simulink model "sm_car"  (R2025a)
settings: Solver=ode23t  StartTime=0.0  StopTime=400  MaxStep=0.4  RelTol=1e-3  AbsTol=1e-3  EnableMultiTasking=on
PreLoadFcn:
  | % Due to usability issue in Repeating Sequence block
  | warning('off','Simulink:Masking:Invalid');
  | 
  | % Eliminate unnecessary warnings in inactive variants
  | % Warnings generated only if you click through inactive variant
  | warning('off','MATLAB:nonExistentField');
  | warning('off','Simulink:Parameters:BlkParamUndefined');
PostLoadFcn:
  | set_param([bdroot '/Vehicle'],'popup_trailer','Off')
  | warning('off','sm:sli:setup:compile:LocalSolverNotSupported')
  | %sm_car_config_maneuver(bdroot,'WOT Braking');
  | sm_car_config_vehicle(bdroot,'false');
  | sm_car_config_logging(bdroot);
InitFcn:
  | sm_car_config_camera;
  | Vehicle = sm_car_vehcfg_checkConfig(Vehicle);
  | sm_car_check_tire_model(bdroot);
StartFcn:
  | tic;
StopFcn:
  | Elapsed_Sim_Time = toc;
  | % disp(['Elapsed Sim Time = ' num2str(Elapsed_Sim_Time)]);
undefined symbols (not defined in the file): Axle1D, AxleIn, Camera, Control, Driver, Free, Init, Maneuver, Pedal, RaceFix, RaceSpin, Scene, ShaftL1, ShaftL2, ShaftR1, ShaftR2, Soft, Stiff, Visual, X, xy_data_car_side, Y, Z
libraries: sm_lib x1546, nesl_utility x528, fl_lib x480, SimscapeFluids_lib x61, sdl_lib x49, simulink x29, ee_lib x7, simulink_extras x6, Linkage_Systems x4, Tire_1x2x x4, AntiRollBar_Systems x2, Linkage_Decoupled x2
(part 6 of 79)

== system sm_car/World/Scene/CRG Hockenheim ==
  Finish Line : Subsystem  mask{post_h=geometry.finish_line.post.height, post_r=geometry.finish_line.post.radius, line_w=geometry.finish_line.post.separation, post_clr=geometry.finish_line.post.clr, post_opc=geometry.finish_line.post.opc, offset_xyz=geometry.finish_line.offset.xyz, offset_yaw=geometry.finish_line.offset.yaw, offset_pitch=geometry.finish_line.offset.pitch, offset_roll=geometry.finish_line.offset.roll}
      mask prompts: post_h "Post Height (m)"; post_r "Post Radius (m)"; line_w "Post Separation (m)"; post_clr "Post Color [R G B] (0-1)"; post_opc "Post Opacity (0-1)"; offset_xyz "Line Offset [x y z] (m)"; offset_yaw "Line Orientation yaw (rad)"; offset_pitch "Line Orientation pitch (rad)"; offset_roll "Line Orientation roll (rad)"
  Ground : Ground
  STL Geometry Centerline : Subsystem  mask{stl_file=geometry.centerline.filename, stl_units=geometry.centerline.fileunits, stl_clr=geometry.centerline.clr, stl_opc=geometry.centerline.opc, stl_x=geometry.centerline.x, stl_y=geometry.centerline.y, stl_z=geometry.centerline.z, stl_yaw=geometry.centerline.yaw, stl_pitch=geometry.centerline.pitch, stl_roll=geometry.centerline.roll}
      mask prompts: stl_file "CAD File"; stl_units "Units"; stl_clr "Color [R G B]"; stl_opc "Opacity (0-1)"; stl_x "Offset x (m)"; stl_y "Offset y (m)"; stl_z "Offset z (m)"; stl_yaw "Offset yaw (rad)"; stl_pitch "Offset pitch (rad)"; stl_roll "Offset roll (rad)"
      mask init:
      | set_param([gcb '/Geometry'],'ExtGeomFileName',stl_file);
      | set_param([gcb '/Geometry'],'ExtGeomFileUnits',stl_units);
  STL Geometry Road : Subsystem  mask{stl_file=geometry.filename, stl_units=geometry.fileunits, stl_clr=geometry.clr, stl_opc=geometry.opc, stl_x=geometry.x, stl_y=geometry.y, stl_z=geometry.z, stl_yaw=geometry.yaw, stl_pitch=geometry.pitch, stl_roll=geometry.roll}
      mask prompts: stl_file "CAD File"; stl_units "Units"; stl_clr "Color [R G B]"; stl_opc "Opacity (0-1)"; stl_x "Offset x (m)"; stl_y "Offset y (m)"; stl_z "Offset z (m)"; stl_yaw "Offset yaw (rad)"; stl_pitch "Offset pitch (rad)"; stl_roll "Offset roll (rad)"
      mask init:
      | set_param([gcb '/Geometry'],'ExtGeomFileName',stl_file);
      | set_param([gcb '/Geometry'],'ExtGeomFileUnits',stl_units);
  W : PMIOPort  Side=Left
  Obs : Outport  VectorParamsAs1DForOutWhenUnconnected=off
  wires:
  Ground/1 -> Obs/1
  connections:
  STL Geometry Centerline/RConn1 -- Finish Line/LConn1 -- W/RConn1 -- STL Geometry Road/RConn1

== system sm_car/World/Scene/CRG Hockenheim F ==
  Finish Line : Subsystem  mask{post_h=geometry.finish_line.post.height, post_r=geometry.finish_line.post.radius, line_w=geometry.finish_line.post.separation, post_clr=geometry.finish_line.post.clr, post_opc=geometry.finish_line.post.opc, offset_xyz=geometry.finish_line.offset.xyz, offset_yaw=geometry.finish_line.offset.yaw, offset_pitch=geometry.finish_line.offset.pitch, offset_roll=geometry.finish_line.offset.roll}
      mask prompts: post_h "Post Height (m)"; post_r "Post Radius (m)"; line_w "Post Separation (m)"; post_clr "Post Color [R G B] (0-1)"; post_opc "Post Opacity (0-1)"; offset_xyz "Line Offset [x y z] (m)"; offset_yaw "Line Orientation yaw (rad)"; offset_pitch "Line Orientation pitch (rad)"; offset_roll "Line Orientation roll (rad)"
  Ground : Ground
  STL Geometry Centerline : Subsystem  mask{stl_file=geometry.centerline.filename, stl_units=geometry.centerline.fileunits, stl_clr=geometry.centerline.clr, stl_opc=geometry.centerline.opc, stl_x=geometry.centerline.x, stl_y=geometry.centerline.y, stl_z=geometry.centerline.z, stl_yaw=geometry.centerline.yaw, stl_pitch=geometry.centerline.pitch, stl_roll=geometry.centerline.roll}
      mask prompts: stl_file "CAD File"; stl_units "Units"; stl_clr "Color [R G B]"; stl_opc "Opacity (0-1)"; stl_x "Offset x (m)"; stl_y "Offset y (m)"; stl_z "Offset z (m)"; stl_yaw "Offset yaw (rad)"; stl_pitch "Offset pitch (rad)"; stl_roll "Offset roll (rad)"
      mask init:
      | set_param([gcb '/Geometry'],'ExtGeomFileName',stl_file);
      | set_param([gcb '/Geometry'],'ExtGeomFileUnits',stl_units);
  STL Geometry Road : Subsystem  mask{stl_file=geometry.filename, stl_units=geometry.fileunits, stl_clr=geometry.clr, stl_opc=geometry.opc, stl_x=geometry.x, stl_y=geometry.y, stl_z=geometry.z, stl_yaw=geometry.yaw, stl_pitch=geometry.pitch, stl_roll=geometry.roll}
      mask prompts: stl_file "CAD File"; stl_units "Units"; stl_clr "Color [R G B]"; stl_opc "Opacity (0-1)"; stl_x "Offset x (m)"; stl_y "Offset y (m)"; stl_z "Offset z (m)"; stl_yaw "Offset yaw (rad)"; stl_pitch "Offset pitch (rad)"; stl_roll "Offset roll (rad)"
      mask init:
      | set_param([gcb '/Geometry'],'ExtGeomFileName',stl_file);
      | set_param([gcb '/Geometry'],'ExtGeomFileUnits',stl_units);
  W : PMIOPort  Side=Left
  Obs : Outport  VectorParamsAs1DForOutWhenUnconnected=off
  wires:
  Ground/1 -> Obs/1
  connections:
  STL Geometry Centerline/RConn1 -- Finish Line/LConn1 -- W/RConn1 -- STL Geometry Road/RConn1

== system sm_car/World/Scene/Plane Grid ==
  Grid : Subsystem  mask{grid_x=plane.l, grid_y=plane.w, grid_z=plane.h, grid_line_width=grid.line_width, grid_num_sq_x=grid.num_sqrs_x, grid_num_sq_y=grid.num_sqrs_y, grid_clr=grid.clr, grid_opc=grid.opc}
      mask prompts: grid_x "Length (m) (Global x)"; grid_y "Width (m) (Global y)"; grid_z "Depth (m) (Global z)"; grid_line_width "Line width (m)"; grid_num_sq_x "Number of squares in x"; grid_num_sq_y "Number of squares in y"; grid_clr "Color [RGB]"; grid_opc "Opacity (0-1)"
      mask init:
      | % Derived parameters - for two perpendicular grids with num_sq-by-1 holes
      | % **Note, not num_sq_x by num_sq_y holes - better render speed with
      | % separate meshes for x and y.
      | 
      | hole_lx = (grid_x-(grid_line_width*(grid_num_sq_x+1)))/grid_num_sq_x;
      | hole_wx = (grid_y-(grid_line_width*(1+1)))/1;
      | 
      | hole_ly = (grid_y-(grid_line_width*(grid_num_sq_y+1)))/grid_num_sq_y;
      | hole_wy = (grid_x-(grid_line_width*(1+1)))/1;
  Ground : Ground
  Ground Plane : Subsystem  mask{gp_l=plane.l, gp_w=plane.w, gp_h=plane.h, gp_clr=plane.clr, gp_opc=plane.opc}
      mask prompts: gp_l "Length (m) (Global  x)"; gp_w "Width (m) (Global  y)"; gp_h "Depth (m) (Global z)"; gp_clr "Color [R G B]"; gp_opc "Opacity (0-1)"
  Transform Plane : sm_lib/Frames and Transforms/Rigid Transform  RotationMethod=None  FollAlignAxisA=+X  BaseAlignAxisA=+Y  FollAlignAxisB=+Y  BaseAlignAxisB=+Z  RotationStandardAxis=+Z  RotationAngle=0.0  RotationAngleUnits=deg  RotationArbitraryAxis=[0 0 1]  RotationSequenceAxes=FollowerAxes  RotationSequence=XYX  RotationSequenceAngles=[0 0 0]  RotationSequenceAnglesUnits=deg  RotationMatrix=[1 0 0; 0 1 0; 0 0 1]  Quaternion=[1 0 0 0]  TranslationMethod=Cartesian  TranslationCartesianOffset=[plane.x plane.y plane.z]  TranslationCartesianOffsetUnits=m  TranslationStandardAxis=+Z  TranslationStandardOffset=0  TranslationStandardOffsetUnits=m  TranslationROffset=0  TranslationROffsetUnits=m  TranslationThetaOffset=0  TranslationThetaOffsetUnits=deg  TranslationZOffset=0  TranslationZOffsetUnits=m
  W : PMIOPort  Side=Left
  Obs : Outport  VectorParamsAs1DForOutWhenUnconnected=off
  wires:
  Ground/1 -> Obs/1
  connections:
  Ground Plane/RConn1 -- Transform Plane/RConn1 -- Grid/LConn1
  Transform Plane/LConn1 -- W/RConn1

== system sm_car/World/Scene/Skidpad ==
  Circle Inner L : Subsystem  mask{circ_d=circ_in.d, circ_a1=-180, circ_a2=180, circ_w=circ_in.w, circ_h=circ_in.h, circ_clr=circ_in.clr, circ_opc=circ_in.opc}
      mask prompts: circ_d "Circle Diameter (m)"; circ_a1 "Start Angle (deg)"; circ_a2 "Finish Angle (deg)"; circ_w "Stripe Width (m)"; circ_h "Stripe Height (m)"; circ_clr "Color [RGB]"; circ_opc "Opacity (0-1)"
      mask init:
      | xy_data_circ = Extr_Data_Ring(...
      |     circ_d/2+circ_w/2,circ_d/2-circ_w/2,circ_a1, circ_a2);
  Circle Inner R : Subsystem  mask{circ_d=circ_in.d, circ_a1=-180, circ_a2=180, circ_w=circ_in.w, circ_h=circ_in.h, circ_clr=circ_in.clr, circ_opc=circ_in.opc}
      mask prompts: circ_d "Circle Diameter (m)"; circ_a1 "Start Angle (deg)"; circ_a2 "Finish Angle (deg)"; circ_w "Stripe Width (m)"; circ_h "Stripe Height (m)"; circ_clr "Color [RGB]"; circ_opc "Opacity (0-1)"
      mask init:
      | xy_data_circ = Extr_Data_Ring(...
      |     circ_d/2+circ_w/2,circ_d/2-circ_w/2,circ_a1, circ_a2);
  Circle Outer L : Subsystem  mask{circ_d=circ_out.d, circ_a1=circ_out.ang1, circ_a2=circ_out.ang2, circ_w=circ_out.w, circ_h=circ_out.h, circ_clr=circ_out.clr, circ_opc=circ_out.opc}
      mask prompts: circ_d "Circle Diameter (m)"; circ_a1 "Start Angle (deg)"; circ_a2 "Finish Angle (deg)"; circ_w "Stripe Width (m)"; circ_h "Stripe Height (m)"; circ_clr "Color [RGB]"; circ_opc "Opacity (0-1)"
      mask init:
      | xy_data_circ = Extr_Data_Ring(...
      |     circ_d/2+circ_w/2,circ_d/2-circ_w/2,circ_a1, circ_a2);
  Circle Outer R : Subsystem  mask{circ_d=circ_out.d, circ_a1=circ_out.ang1, circ_a2=circ_out.ang2, circ_w=circ_out.w, circ_h=circ_out.h, circ_clr=circ_out.clr, circ_opc=circ_out.opc}
      mask prompts: circ_d "Circle Diameter (m)"; circ_a1 "Start Angle (deg)"; circ_a2 "Finish Angle (deg)"; circ_w "Stripe Width (m)"; circ_h "Stripe Height (m)"; circ_clr "Color [RGB]"; circ_opc "Opacity (0-1)"
      mask init:
      | xy_data_circ = Extr_Data_Ring(...
      |     circ_d/2+circ_w/2,circ_d/2-circ_w/2,circ_a1, circ_a2);
  Ground : Ground
  Ground Plane : Subsystem  mask{gp_l=plane.l, gp_w=plane.w, gp_h=plane.h, gp_clr=plane.clr, gp_opc=plane.opc}
      mask prompts: gp_l "Length (m) (Global  x)"; gp_w "Width (m) (Global  y)"; gp_h "Depth (m) (Global z)"; gp_clr "Color [R G B]"; gp_opc "Opacity (0-1)"
  Transform Circle L : sm_lib/Frames and Transforms/Rigid Transform  RotationMethod=None  FollAlignAxisA=+X  BaseAlignAxisA=+Y  FollAlignAxisB=+Y  BaseAlignAxisB=+Z  RotationStandardAxis=+Z  RotationAngle=0.0  RotationAngleUnits=deg  RotationArbitraryAxis=[0 0 1]  RotationSequenceAxes=FollowerAxes  RotationSequence=XYX  RotationSequenceAngles=[0 0 0]  RotationSequenceAnglesUnits=deg  RotationMatrix=[1 0 0; 0 1 0; 0 0 1]  Quaternion=[1 0 0 0]  TranslationMethod=Cartesian  TranslationCartesianOffset=[0 circ_in.sep/2 0]  TranslationCartesianOffsetUnits=m  TranslationStandardAxis=+Z  TranslationStandardOffset=0  TranslationStandardOffsetUnits=m  TranslationROffset=0  TranslationROffsetUnits=m  TranslationThetaOffset=0  TranslationThetaOffsetUnits=deg  TranslationZOffset=0  TranslationZOffsetUnits=m
  Transform Circle R : sm_lib/Frames and Transforms/Rigid Transform  RotationMethod=None  FollAlignAxisA=+X  BaseAlignAxisA=+Y  FollAlignAxisB=+Y  BaseAlignAxisB=+Z  RotationStandardAxis=+Z  RotationAngle=0.0  RotationAngleUnits=deg  RotationArbitraryAxis=[0 0 1]  RotationSequenceAxes=FollowerAxes  RotationSequence=XYX  RotationSequenceAngles=[0 0 0]  RotationSequenceAnglesUnits=deg  RotationMatrix=[1 0 0; 0 1 0; 0 0 1]  Quaternion=[1 0 0 0]  TranslationMethod=Cartesian  TranslationCartesianOffset=[0 -circ_in.sep/2 0]  TranslationCartesianOffsetUnits=m  TranslationStandardAxis=+Z  TranslationStandardOffset=0  TranslationStandardOffsetUnits=m  TranslationROffset=0  TranslationROffsetUnits=m  TranslationThetaOffset=0  TranslationThetaOffsetUnits=deg  TranslationZOffset=0  TranslationZOffsetUnits=m
  Transform Orient OuterL : sm_lib/Frames and Transforms/Rigid Transform  RotationMethod=StandardAxis  FollAlignAxisA=+X  BaseAlignAxisA=+Y  FollAlignAxisB=+Y  BaseAlignAxisB=+Z  RotationStandardAxis=+Z  RotationAngle=90  RotationAngleUnits=deg  RotationArbitraryAxis=[0 0 1]  RotationSequenceAxes=FollowerAxes  RotationSequence=XYX  RotationSequenceAngles=[0 0 0]  RotationSequenceAnglesUnits=deg  RotationMatrix=[1 0 0; 0 1 0; 0 0 1]  Quaternion=[1 0 0 0]  TranslationMethod=None  TranslationCartesianOffset=[0 0 0]  TranslationCartesianOffsetUnits=m  TranslationStandardAxis=+Z  TranslationStandardOffset=0  TranslationStandardOffsetUnits=m  TranslationROffset=0  TranslationROffsetUnits=m  TranslationThetaOffset=0  TranslationThetaOffsetUnits=deg  TranslationZOffset=0  TranslationZOffsetUnits=m
  Transform Orient OuterR : sm_lib/Frames and Transforms/Rigid Transform  RotationMethod=StandardAxis  FollAlignAxisA=+X  BaseAlignAxisA=+Y  FollAlignAxisB=+Y  BaseAlignAxisB=+Z  RotationStandardAxis=+Z  RotationAngle=-90  RotationAngleUnits=deg  RotationArbitraryAxis=[0 0 1]  RotationSequenceAxes=FollowerAxes  RotationSequence=XYX  RotationSequenceAngles=[0 0 0]  RotationSequenceAnglesUnits=deg  RotationMatrix=[1 0 0; 0 1 0; 0 0 1]  Quaternion=[1 0 0 0]  TranslationMethod=None  TranslationCartesianOffset=[0 0 0]  TranslationCartesianOffsetUnits=m  TranslationStandardAxis=+Z  TranslationStandardOffset=0  TranslationStandardOffsetUnits=m  TranslationROffset=0  TranslationROffsetUnits=m  TranslationThetaOffset=0  TranslationThetaOffsetUnits=deg  TranslationZOffset=0  TranslationZOffsetUnits=m
  Transform Plane : sm_lib/Frames and Transforms/Rigid Transform  RotationMethod=None  FollAlignAxisA=+X  BaseAlignAxisA=+Y  FollAlignAxisB=+Y  BaseAlignAxisB=+Z  RotationStandardAxis=+Z  RotationAngle=0.0  RotationAngleUnits=deg  RotationArbitraryAxis=[0 0 1]  RotationSequenceAxes=FollowerAxes  RotationSequence=XYX  RotationSequenceAngles=[0 0 0]  RotationSequenceAnglesUnits=deg  RotationMatrix=[1 0 0; 0 1 0; 0 0 1]  Quaternion=[1 0 0 0]  TranslationMethod=Cartesian  TranslationCartesianOffset=[plane.x plane.y plane.z]  TranslationCartesianOffsetUnits=m  TranslationStandardAxis=+Z  TranslationStandardOffset=0  TranslationStandardOffsetUnits=m  TranslationROffset=0  TranslationROffsetUnits=m  TranslationThetaOffset=0  TranslationThetaOffsetUnits=deg  TranslationZOffset=0  TranslationZOffsetUnits=m
  W : PMIOPort  Side=Left
  Obs : Outport  VectorParamsAs1DForOutWhenUnconnected=off
  wires:
  Ground/1 -> Obs/1
  connections:
  Circle Outer L/RConn1 -- Transform Orient OuterL/RConn1
  Circle Outer R/RConn1 -- Transform Orient OuterR/RConn1
  Circle Inner R/RConn1 -- Transform Circle R/RConn1 -- Transform Orient OuterR/LConn1
  Transform Plane/RConn1 -- Ground Plane/RConn1
  Transform Circle L/LConn1 -- W/RConn1 -- Transform Plane/LConn1 -- Transform Circle R/LConn1
  Circle Inner L/RConn1 -- Transform Circle L/RConn1 -- Transform Orient OuterL/LConn1

== system sm_car/World/Visuals/Off ==
  Reference Frame : sm_lib/Frames and Transforms/Reference Frame
  W : PMIOPort  Side=Left
  connections:
  Reference Frame/RConn1 -- W/RConn1

== system sm_car/Controller/Default/Brake Control/Pedal ==
  rBrakePedal : Inport
  VehBus : Inport  Port=2
  Apply{,1..3} (4 alike) : Constant  Value=[0 1]
  Bus Creator : BusCreator  Inputs=1
  Bus Creator1 : BusCreator  Inputs=4
  Terminator : Terminator
  Terminator1 : Terminator
  Brakes : Outport  VectorParamsAs1DForOutWhenUnconnected=off
  wires:
  rBrakePedal/1 -> Terminator1/1
  Apply3/1 -> Bus Creator1/4  "R2"
  Apply2/1 -> Bus Creator1/3  "L2"
  Apply1/1 -> Bus Creator1/2  "R1"
  Apply/1 -> Bus Creator1/1  "L1"
  Bus Creator1/1 -> Bus Creator/1  "Valves"
  VehBus/1 -> Terminator/1
  Bus Creator/1 -> Brakes/1  "Brakes"

== system sm_car/Controller/Default/Damper Control/Damper Control A1 ==
  mL : Inport
  mR : Inport  Port=2
  Inp : Inport  Port=3
  None : Subsystem  VariantControl=None
  L : Outport
  R : Outport  Port=2

== system sm_car/Controller/Default/Damper Control/Damper Control A2 ==
  mL : Inport
  mR : Inport  Port=2
  Inp : Inport  Port=3
  None : Subsystem  VariantControl=None
  L : Outport
  R : Outport  Port=2

== system sm_car/Controller/Default/Spring Control/Spring Control A1 ==
  mL : Inport
  mR : Inport  Port=2
  Inp : Inport  Port=3
  Hydropneumatic : Subsystem  VariantControl=Hydropneumatic  mask{popup_gas_spring=Soft}
      mask prompts: popup_gas_spring "Gas Spring"
      mask init:
      | bh = gcb;
      | popup_gas_spring_str = get_param(bh,'popup_gas_spring');
      | 
      | if(strcmp(popup_gas_spring_str,'Stiff'))
      |     soft_suspension = 0;
      | elseif(strcmp(popup_gas_spring_str,'Soft'))
      |     soft_suspension = 1;
      | end
      mask TypeOptions popup_gas_spring: Stiff | Soft
  None : Subsystem  VariantControl=None
  L : Outport  VectorParamsAs1DForOutWhenUnconnected=off
  R : Outport  Port=2  VectorParamsAs1DForOutWhenUnconnected=off

== system sm_car/Controller/Default/Spring Control/Spring Control A2 ==
  mL : Inport
  mR : Inport  Port=2
  Inp : Inport  Port=3
  Hydropneumatic : Subsystem  VariantControl=Hydropneumatic  mask{popup_gas_spring=Soft}
      mask prompts: popup_gas_spring "Gas Spring"
      mask init: same as sm_car/Controller/Default/Spring Control/Spring Control A1/Hydropneumatic
      mask TypeOptions popup_gas_spring: Stiff | Soft
  None : Subsystem  VariantControl=None
  L : Outport  VectorParamsAs1DForOutWhenUnconnected=off
  R : Outport  Port=2  VectorParamsAs1DForOutWhenUnconnected=off

== system sm_car/Controller/Default/Susp/Steer Axle 1 ==
  note: Example Steer by Wire algorithm.
      | Used by steering models where rack position
      | and steering wheel angle inputs are both used.
  aSteerWheel : Inport
  vx : Inport  Port=2
  Bus Creator4 : BusCreator  Inputs=2
  Product1 : Product
  Transfer Fcn (with initial states)1 : simulink_extras/Additional Linear/Transfer Fcn (with initial states)  N=[1]  D="[1/Steer.fActuatorCutoff.Value  1]"  X0=-1
  Vehicle Speed to Ratio Scale : Lookup_n-D  NumberOfTableDimensions=1  BreakpointsForDimension1=Control.Default.Steer.Ratio_Scale.vVehicle.Value  Table=Control.Default.Steer.Ratio_Scale.n.Value  InternalRulePriority=Speed  RndMeth=Simplest
  Wheel Angle to Steer Ratio : Lookup_n-D  NumberOfTableDimensions=1  BreakpointsForDimension1=Control.Default.Steer.Ratio_Table.aWheel.Value  Table=Control.Default.Steer.Ratio_Table.xRack.Value  InternalRulePriority=Speed  RndMeth=Simplest
  Steer : Outport  VectorParamsAs1DForOutWhenUnconnected=off
  wires:
  Vehicle Speed to Ratio Scale/1 -> Product1/1  "nRatioScale"
  Transfer Fcn (with initial states)1/1 -> Vehicle Speed to Ratio Scale/1
  aSteerWheel/1 -> Wheel Angle to Steer Ratio/1, Bus Creator4/2  "aSteerWheel"
  Wheel Angle to Steer Ratio/1 -> Product1/2  "xRack"
  Product1/1 -> Bus Creator4/1  "xRack"
  vx/1 -> Transfer Fcn (with initial states)1/1
  Bus Creator4/1 -> Steer/1  "Steer"

== system sm_car/Controller/Default/Susp/Steer Axle 2 ==
  note: Example rear steer algorithm
      | Rack position is based on steering wheel angle
      | and is scaled based on vehicle speed.
  aSteerWheel : Inport
  vx : Inport  Port=2
  1-D Lookup Table : Lookup_n-D  NumberOfTableDimensions=1  BreakpointsForDimension1=Steer.Gain.vVehicle.Value  Table=Steer.Gain.n.Value  InterpMethod=Linear Lagrange  InternalRulePriority=Speed  RndMeth=Simplest
  Bus Creator2 : BusCreator  Inputs=2
  Filter : simulink_extras/Additional Linear/Transfer Fcn (with initial states)  N=[1]  D="[1/Steer.fActuatorCutoff.Value  1]"  X0=-1
  Gain : Gain  Gain=3.6
  Gain1 : Gain  Gain=Steer.Gain.nRearAct.Value
  Product : Product
  Saturation : Saturate  UpperLimit=Steer.Limits.aUpper.Value  LowerLimit=Steer.Limits.aLower.Value  LinearizeAsGain=off  ZeroCross=off
  Steer : Outport
  wires:
  aSteerWheel/1 -> Product/1
  Gain/1 -> 1-D Lookup Table/1
  Bus Creator2/1 -> Steer/1  "Steer"
  Saturation/1 -> Bus Creator2/1, Gain1/1  "aSteerWheel"
  Product/1 -> Saturation/1
  Filter/1 -> Product/2
  Gain1/1 -> Bus Creator2/2  "xSteerActuator"
  1-D Lookup Table/1 -> Filter/1
  vx/1 -> Gain/1

== system sm_car/Controller/TrqVec 4Motor/Brake Control/ABS ==
  rBrakePedal : Inport
  In Bus Element1 : Inport  Port=2  PortName=VehBus  Element=Chassis
  In Bus Element2 : Inport  Port=2  PortName=VehBus  Element=Chassis.Body.CG
  Bus Creator1 : BusCreator  Inputs=4
  Bus Creator2 : BusCreator  Inputs=1
  Bus Selector : BusSelector  OutputSignals=L1
  Bus Selector1 : BusSelector  OutputSignals=R1
  Bus Selector2 : BusSelector  OutputSignals=L2
  Bus Selector3 : BusSelector  OutputSignals=R2
  Calculate Slip : Subsystem
  Sensor : Subsystem
  Terminator : Terminator
  Valve Control L1 : Subsystem
  Valve Control L2 : Subsystem
  Valve Control R1 : Subsystem
  Valve Control R2 : Subsystem
  Vehicle Speed : Subsystem
  Brakes : Outport  VectorParamsAs1DForOutWhenUnconnected=off
  wires:
  rBrakePedal/1 -> Terminator/1
  Vehicle Speed/1(vSpdEst) -> Valve Control R2/2(vSpdEst), Valve Control L2/2(vSpdEst), Valve Control R1/2(vSpdEst), Valve Control L1/2(vSpdEst), Calculate Slip/2(VehSpdEst)
  Sensor/1(GroundSpd) -> Vehicle Speed/1(Sensors), Calculate Slip/1(WhlSpd)
  Bus Creator1/1 -> Bus Creator2/1  "Valves"
  Bus Selector2/1 -> Valve Control L2/1(Slip)  "<L2>"
  Valve Control R1/1(Valve) -> Bus Creator1/2  "R1"
  Valve Control R2/1(Valve) -> Bus Creator1/4  "R2"
  Valve Control L2/1(Valve) -> Bus Creator1/3  "L2"
  Bus Selector3/1 -> Valve Control R2/1(Slip)  "<R2>"
  Bus Selector/1 -> Valve Control L1/1(Slip)  "<L1>"
  Calculate Slip/1(Slip) -> Bus Selector3/1, Bus Selector2/1, Bus Selector1/1, Bus Selector/1
  Valve Control L1/1(Valve) -> Bus Creator1/1  "L1"
  Bus Selector1/1 -> Valve Control R1/1(Slip)  "<R1>"
  Bus Creator2/1 -> Brakes/1  "Brakes"
  In Bus Element1/1 -> Sensor/2(WhlSpd)
  In Bus Element2/1 -> Sensor/1(Body)

== system sm_car/Controller/TrqVec 4Motor/Brake Control/Pedal ==
  rBrakePedal : Inport
  VehBus : Inport  Port=2
  Apply{,1..3} (4 alike) : Constant  Value=[0 1]
  Bus Creator : BusCreator  Inputs=1
  Bus Creator1 : BusCreator  Inputs=4
  Terminator : Terminator
  Terminator1 : Terminator
  Brakes : Outport  VectorParamsAs1DForOutWhenUnconnected=off
  wires:
  rBrakePedal/1 -> Terminator1/1
  Apply3/1 -> Bus Creator1/4  "R2"
  Apply2/1 -> Bus Creator1/3  "L2"
  Apply1/1 -> Bus Creator1/2  "R1"
  Apply/1 -> Bus Creator1/1  "L1"
  Bus Creator1/1 -> Bus Creator/1  "Valves"
  VehBus/1 -> Terminator/1
  Bus Creator/1 -> Brakes/1  "Brakes"

== system sm_car/Controller/TrqVec 4Motor/Brake Control/Pressure ==
  rBrakePedal : Inport
  VehBus : Inport  Port=2
  Bus Creator : BusCreator  Inputs=4
  Gain : Gain  Gain=Vehicle.Brakes.Front.Caliper.pMax.Value
  Gain1 : Gain  Gain=Vehicle.Brakes.Front.Caliper.pMax.Value
  Gain2 : Gain  Gain=Vehicle.Brakes.Rear.Caliper.pMax.Value
  Gain3 : Gain  Gain=Vehicle.Brakes.Rear.Caliper.pMax.Value
  Terminator : Terminator
  Brakes : Outport  VectorParamsAs1DForOutWhenUnconnected=off
  wires:
  rBrakePedal/1 -> Gain/1, Gain1/1, Gain3/1, Gain2/1
  VehBus/1 -> Terminator/1
  Bus Creator/1 -> Brakes/1  "Brakes"
  Gain/1 -> Bus Creator/1  "pBrakeL1"
  Gain1/1 -> Bus Creator/2  "pBrakeR1"
  Gain2/1 -> Bus Creator/3  "pBrakeL2"
  Gain3/1 -> Bus Creator/4  "pBrakeR2"

== system sm_car/Controller/TrqVec 4Motor/Damper Control/Damper Control A1 ==
  mL : Inport
  mR : Inport  Port=2
  Inp : Inport  Port=3
  Coefficient : Subsystem  VariantControl=Coefficient  mask(Control Law for Damper Coefficient){b_A1=ControlDamper.tFilt, brkPts_dim1_A1=ControlDamper.vDamperd, brkPts_dim2_A1=ControlDamper.iControl, Table_A1=ControlDamper.dDamper}
      mask prompts: b_A1 "Filter time constant (sec)"; brkPts_dim1_A1 "Damper Speed [1xm] (m/s)"; brkPts_dim2_A1 "Input 2 [1xn] (1)"; Table_A1 "Damper Coefficient [mxn] (N/(m/s))"
      mask help: Determines damping coefficient based on damper speed and a second input signal.
      mask TypeOptions b_A1: Filter/b
      mask TypeOptions brkPts_dim1_A1: Lookup Table Coeff/BreakpointsForDimension1
      mask TypeOptions brkPts_dim2_A1: Lookup Table Coeff/BreakpointsForDimension2
      mask TypeOptions Table_A1: Lookup Table Coeff/Table
      mask DialogControl cont_axle1 Prompt: Axle 1
  Force : Subsystem  VariantControl=Force  mask(Control Law for Damper Force){b_A1=ControlDamper.tFilt, brkPts_dim1_A1=ControlDamper.vDamperf, brkPts_dim2_A1=ControlDamper.iControl, Table_A1=ControlDamper.fDamper}
      mask prompts: b_A1 "Filter time constant (sec)"; brkPts_dim1_A1 "Damper Speed [1xm] (m/s)"; brkPts_dim2_A1 "Input 2 [1xn] (1)"; Table_A1 "Damper Force [mxn] (N)"
      mask help: Determines damping force based on damper speed and a second input signal.
      mask TypeOptions b_A1: Filter/b
      mask TypeOptions brkPts_dim1_A1: Lookup Table A1/BreakpointsForDimension1
      mask TypeOptions brkPts_dim2_A1: Lookup Table A1/BreakpointsForDimension2
      mask TypeOptions Table_A1: Lookup Table A1/Table
      mask DialogControl cont_axle1 Prompt: Axle 1
  None : Subsystem  VariantControl=None
  L : Outport
  R : Outport  Port=2

== system sm_car/Controller/TrqVec 4Motor/Damper Control/Damper Control A2 ==
  mL : Inport
  mR : Inport  Port=2
  Inp : Inport  Port=3
  Coefficient : Subsystem  VariantControl=Coefficient  mask(Control Law for Damper Coefficient){b_A1=ControlDamper.tFilt, brkPts_dim1_A1=ControlDamper.vDamperd, brkPts_dim2_A1=ControlDamper.iControl, Table_A1=ControlDamper.dDamper}
      mask prompts: b_A1 "Filter time constant (sec)"; brkPts_dim1_A1 "Damper Speed [1xm] (m/s)"; brkPts_dim2_A1 "Input 2 [1xn] (1)"; Table_A1 "Damper Coefficient [mxn] (N/(m/s))"
      mask help: Determines damping coefficient based on damper speed and a second input signal.
      mask TypeOptions b_A1: Filter/b
      mask TypeOptions brkPts_dim1_A1: Lookup Table Coeff/BreakpointsForDimension1
      mask TypeOptions brkPts_dim2_A1: Lookup Table Coeff/BreakpointsForDimension2
      mask TypeOptions Table_A1: Lookup Table Coeff/Table
      mask DialogControl cont_axle1 Prompt: Axle 1
  Force : Subsystem  VariantControl=Force  mask(Control Law for Damper Force){b_A1=ControlDamper.tFilt, brkPts_dim1_A1=ControlDamper.vDamperf, brkPts_dim2_A1=ControlDamper.iControl, Table_A1=ControlDamper.fDamper}
      mask prompts: b_A1 "Filter time constant (sec)"; brkPts_dim1_A1 "Damper Speed [1xm] (m/s)"; brkPts_dim2_A1 "Input 2 [1xn] (1)"; Table_A1 "Damper Force [mxn] (N)"
      mask help: Determines damping force based on damper speed and a second input signal.
      mask TypeOptions b_A1: Filter/b
      mask TypeOptions brkPts_dim1_A1: Lookup Table A1/BreakpointsForDimension1
      mask TypeOptions brkPts_dim2_A1: Lookup Table A1/BreakpointsForDimension2
      mask TypeOptions Table_A1: Lookup Table A1/Table
      mask DialogControl cont_axle1 Prompt: Axle 1
  None : Subsystem  VariantControl=None
  L : Outport
  R : Outport  Port=2

== system sm_car/Controller/TrqVec 4Motor/Power_TqVec/Torque Vectoring ==
  trqA2 : Inport
  vx : Inport  Port=2
  aSteerWheel : Inport  Port=3
  wL2 : Inport  Port=4
  wR2 : Inport  Port=5
  nYaw : Inport  Port=6
  rBrake : Inport  Port=7
  Accel Torque Request : Subsystem
  Calculate Torque Split : MATLAB Function  TreatAsAtomicUnit=on
  Compare To Constant1 : simulink/Logic and Bit Operations/Compare To Constant  relop=<  const=.01  OutDataTypeStr=boolean
  Data Type Conversion : DataTypeConversion  SaturateOnIntegerOverflow=off  RndMeth=Floor
  Enable : Subsystem
  Gain1 : Gain  Gain=0.5
  Gain5 : Gain
  Gain6 : Gain
  Max Delta Torque : Constant  Value=max_torque_delta
  PID Controller : slpidlib/PID Controller  Controller=PID  Form=Parallel  TimeDomain=Continuous-time  UseExternalTs=off  SampleTime=-1  IntegratorMethod=Forward Euler  FilterMethod=Forward Euler  ControllerParametersSource=internal  P=P  I=I  UseKiTs=off  D=0  UseExternalDerivativeSource=off  N=1  UseFilter=on  TunerSelectOption=Transfer Function Based (PID Tuner App)  InitialConditionSource=internal  InitialConditionForIntegrator=0  InitialConditionForFilter=0  DifferentiatorICPrevScaledInput=0  ExternalReset=either  TrackingMode=off  Kt=1  LimitOutput=off  SatLimitsSource=internal  UpperSaturationLimit=inf  LowerSaturationLimit=-inf  LinearizeAsGain=on  AntiWindupMode=back-calculation  Kb=1  LimitIntegrator=off  UpperIntegratorSaturationLimit=inf  LowerIntegratorSaturationLimit=-inf  POutMin=[]  POutMax=[]  IOutMin=[]  IOutMax=[]  DOutMin=[]  DOutMax=[]  NOutMin=[]  NOutMax=[]  SumOutMin=[]  SumOutMax=[]  SaturationOutMin=[]  SaturationOutMax=[]  PParamMin=[]  PParamMax=[]  IParamMin=[]  IParamMax=[]  DParamMin=[]  DParamMax=[]  NParamMin=[]  NParamMax=[]  KbParamMin=[]  KbParamMax=[]  KtParamMin=[]  KtParamMax=[]  KbOutMin=[]  KbOutMax=[]  KtOutMin=[]  KtOutMax=[]  IntegratorOutMin=[]  IntegratorOutMax=[]  FilterOutMin=[]  FilterOutMax=[]  SumI1OutMin=[]  SumI1OutMax=[]  SumI2OutMin=[]  SumI2OutMax=[]  SumI3OutMin=[]  SumI3OutMax=[]  SumI4OutMin=[]  SumI4OutMax=[]  SumDOutMin=[]  SumDOutMax=[]  DifferentiatorOutMin=[]  DifferentiatorOutMax=[]  FilterDiffOutCoefMin=[]  FilterDiffOutCoefMax=[]  ReciprocalOutMin=[]  ReciprocalOutMax=[]  SumDenOutMin=[]  SumDenOutMax=[]  SumNumOutMin=[]  SumNumOutMax=[]  DivideOutMin=[]  DivideOutMax=[]  UdiffTsProdOutMin=[]  UdiffTsProdOutMax=[]  NTsProdOutMin=[]  NTsProdOutMax=[]  UintegralTsProdOutMin=[]  UintegralTsProdOutMax=[]  UngainTsProdOutMin=[]  UngainTsProdOutMax=[]  ClampingZeroOutDataTypeStr=Inherit: Inherit via back propagation  ClampingZeroOutMin=[]  ClampingZeroOutMax=[]  FilterDenConstantOutDataTypeStr=Inherit: Inherit via back propagation  FilterDenConstantOutMin=[]  FilterDenConstantOutMax=[]  PCopyOutDataTypeStr=Inherit: Inherit via back propagation  PCopyOutMin=[]  PCopyOutMax=[]  NCopyOutDataTypeStr=Inherit: Inherit via back propagation  NCopyOutMin=[]  NCopyOutMax=[]  IntegratorContinuousStateAttributes=''  IntegratorStateMustResolveToSignalObject=off  IntegratorRTWStateStorageClass=Auto  FilterContinuousStateAttributes=''  FilterStateMustResolveToSignalObject=off  FilterRTWStateStorageClass=Auto  ParallelPVariant=InternalParameters  IdealPVariant=Disabled  IVariant=InternalParameters  DVariant=InternalParameters  IntegratorVariant=Continuous  SatVariant=Disabled  AWVariant=Passthrough  PCopyVariant=Disabled  TRVariant=Disabled  FdbkBlocksVariant=Forward  IdealPFdbkVariant=Disabled  SatFdbkVariant=Disabled  DerivativeFilterVariant=ContFilter  NVariant=InternalParameters  NCopyVariant=Disabled  FilterICVariant=InternalICsFilter  IntegratorICVariant=InternalICs  ExternalResetVariant=ExternalReset  TRSumVariant=Passthrough  SumFdbkVariant=Disabled  SumVariant=Sum_PID  TsampFilterVariant=InternalTs  TsampNgainVariant=Passthrough  TsampIntegralVariant=Disabled_SignalSpec  ExternalSaturationOutDataTypeStr=Inherit: Same as second input  DerivativeSourceVariant=ErrorSignal  PreIntVariant=InternalPreInt
  Transfer Fcn : TransferFcn  Denominator=[0.5 1]
  Transfer Fcn1 : TransferFcn  Denominator=[.001 1]
  Transfer Fcn2 : TransferFcn  Denominator=[.001 1]
  Vehicle Slip Angle Error : Subsystem
  trqL2 : Outport  VectorParamsAs1DForOutWhenUnconnected=off
  trqR2 : Outport  Port=2  VectorParamsAs1DForOutWhenUnconnected=off
  wires:
  Compare To Constant1/1 -> Data Type Conversion/1
  Data Type Conversion/1 -> Transfer Fcn/1
  Max Delta Torque/1 -> Calculate Torque Split/2(max_delta_trq)
  nYaw/1 -> Vehicle Slip Angle Error/3(nYaw)
  Enable/1(Enable) -> Calculate Torque Split/1(enable), PID Controller/2  "Enable"
  Gain1/1 -> Calculate Torque Split/4(tq_l), Calculate Torque Split/5(tq_r)
  rBrake/1 -> Compare To Constant1/1
  Gain6/1 -> trqR2/1
  Vehicle Slip Angle Error/1(Error) -> PID Controller/1
  Calculate Torque Split/1(tq_l_out) -> Gain5/1
  Transfer Fcn/1 -> Calculate Torque Split/7(brk)
  Transfer Fcn2/1 -> Accel Torque Request/2(MotSpdR2)
  trqA2/1 -> Gain1/1
  Calculate Torque Split/2(tq_r_out) -> Gain6/1
  wR2/1 -> Transfer Fcn2/1
  PID Controller/1 -> Calculate Torque Split/6(tq_tv)
  Gain5/1 -> trqL2/1
  aSteerWheel/1 -> Enable/2(aSteerWheel), Vehicle Slip Angle Error/2(aSteerWheel)
  vx/1 -> Enable/1(vx), Vehicle Slip Angle Error/1(vx)
  Accel Torque Request/1(TrqMax) -> Calculate Torque Split/3(max_tq)
  Transfer Fcn1/1 -> Accel Torque Request/1(MotSpdL2)
  wL2/1 -> Transfer Fcn1/1

== system sm_car/Controller/TrqVec 4Motor/Spring Control/Spring Control A1 ==
  mL : Inport
  mR : Inport  Port=2
  Inp : Inport  Port=3
  Hydropneumatic : Subsystem  VariantControl=Hydropneumatic  mask{popup_gas_spring=Stiff}
      mask prompts: popup_gas_spring "Gas Spring"
      mask init: same as sm_car/Controller/Default/Spring Control/Spring Control A1/Hydropneumatic
      mask TypeOptions popup_gas_spring: Stiff | Soft
  None : Subsystem  VariantControl=None
  L : Outport  VectorParamsAs1DForOutWhenUnconnected=off
  R : Outport  Port=2  VectorParamsAs1DForOutWhenUnconnected=off

== system sm_car/Controller/TrqVec 4Motor/Spring Control/Spring Control A2 ==
  mL : Inport
  mR : Inport  Port=2
  Inp : Inport  Port=3
  Hydropneumatic : Subsystem  VariantControl=Hydropneumatic  mask{popup_gas_spring=Stiff}
      mask prompts: popup_gas_spring "Gas Spring"
      mask init: same as sm_car/Controller/Default/Spring Control/Spring Control A1/Hydropneumatic
      mask TypeOptions popup_gas_spring: Stiff | Soft
  None : Subsystem  VariantControl=None
  L : Outport  VectorParamsAs1DForOutWhenUnconnected=off
  R : Outport  Port=2  VectorParamsAs1DForOutWhenUnconnected=off

== system sm_car/Controller/TrqVec 4Motor/Susp/Steer Axle 1 ==
  note: Example Steer by Wire algorithm.
      | Used by steering models where rack position
      | and steering wheel angle inputs are both used.
  aSteerWheel : Inport
  vx : Inport  Port=2
  Bus Creator4 : BusCreator  Inputs=2
  Product1 : Product
  Transfer Fcn (with initial states)1 : simulink_extras/Additional Linear/Transfer Fcn (with initial states)  N=[1]  D="[1/Steer.fActuatorCutoff.Value  1]"  X0=-1
  Vehicle Speed to Ratio Scale : Lookup_n-D  NumberOfTableDimensions=1  BreakpointsForDimension1=Control.Default.Steer.Ratio_Scale.vVehicle.Value  Table=Control.Default.Steer.Ratio_Scale.n.Value  InternalRulePriority=Speed  RndMeth=Simplest
  Wheel Angle to Steer Ratio : Lookup_n-D  NumberOfTableDimensions=1  BreakpointsForDimension1=Control.Default.Steer.Ratio_Table.aWheel.Value  Table=Control.Default.Steer.Ratio_Table.xRack.Value  InternalRulePriority=Speed  RndMeth=Simplest
  Steer : Outport  VectorParamsAs1DForOutWhenUnconnected=off
  wires:
  Vehicle Speed to Ratio Scale/1 -> Product1/1  "nRatioScale"
  Transfer Fcn (with initial states)1/1 -> Vehicle Speed to Ratio Scale/1
  aSteerWheel/1 -> Wheel Angle to Steer Ratio/1, Bus Creator4/2  "aSteerWheel"
  Wheel Angle to Steer Ratio/1 -> Product1/2  "xRack"
  Product1/1 -> Bus Creator4/1  "xRack"
  vx/1 -> Transfer Fcn (with initial states)1/1
  Bus Creator4/1 -> Steer/1  "Steer"

== system sm_car/Controller/TrqVec 4Motor/Susp/Steer Axle 2 ==
  note: Example rear steer algorithm
      | Rack position is based on steering wheel angle
      | and is scaled based on vehicle speed.
  aSteerWheel : Inport
  vx : Inport  Port=2
  1-D Lookup Table : Lookup_n-D  NumberOfTableDimensions=1  BreakpointsForDimension1=Steer.Gain.vVehicle.Value  Table=Steer.Gain.n.Value  InterpMethod=Linear Lagrange  InternalRulePriority=Speed  RndMeth=Simplest
  Bus Creator2 : BusCreator  Inputs=2
  Filter : simulink_extras/Additional Linear/Transfer Fcn (with initial states)  N=[1]  D="[1/Steer.fActuatorCutoff.Value  1]"  X0=-1
  Gain : Gain  Gain=3.6
  Gain1 : Gain  Gain=Steer.Gain.nRearAct.Value
  Product : Product
  Saturation : Saturate  UpperLimit=Steer.Limits.aUpper.Value  LowerLimit=Steer.Limits.aLower.Value  LinearizeAsGain=off  ZeroCross=off
  Steer : Outport
  wires:
  aSteerWheel/1 -> Product/1
  Gain/1 -> 1-D Lookup Table/1
  Bus Creator2/1 -> Steer/1  "Steer"
  Saturation/1 -> Bus Creator2/1, Gain1/1  "aSteerWheel"
  Product/1 -> Saturation/1
  Filter/1 -> Product/2
  Gain1/1 -> Bus Creator2/2  "xSteerActuator"
  1-D Lookup Table/1 -> Filter/1
  vx/1 -> Gain/1

== system sm_car/Driver/Closed Loop/Driver/Cur Pose ==
  Cur : Inport
  Demux : Demux  Outputs=3
  Gain : Gain  Gain=pi/180
  Mux : Mux  Inputs=3
  CurPose : Outport  VectorParamsAs1DForOutWhenUnconnected=off
  wires:
  Gain/1 -> Mux/3
  Demux/3 -> Gain/1
  Demux/2 -> Mux/2
  Mux/1 -> CurPose/1
  Cur/1 -> Demux/1
  Demux/1 -> Mux/1

== system sm_car/Driver/Closed Loop/Driver/Fwd Rev ==
  note: This logic enables the driver models to handle maneuvers where the vehicle is driven in reverse.
  note: When driving in reverse, swap sign so that only positive velocities are fed to Longitudinal Driver model.
  vx : Inport
  vT : Inport  Port=2
  Product : Product
  Sign : Signum  ZeroCross=off
  dir : Outport
  vxFwRv : Outport  Port=2
  wires:
  Product/1 -> vxFwRv/1
  vx/1 -> Product/1
  Sign/1 -> Product/2, dir/1  "Direction"
  vT/1 -> Sign/1

== system sm_car/Driver/Closed Loop/Driver/Lateral Driver ==
  referencePose : Inport
  Distance : Inport  Port=2
  currentPose : Inport  Port=3
  v_x : Inport  Port=4
  Preview : Inport  Port=5
  Direction : Inport  Port=6
  Pure Pursuit : Subsystem  VariantControl=Pure_Pursuit  mask(Lateral Driver (Pure Pursuit)){MAX_STEERING_ANGLE_DEG=Lateral.aMaxSteer.Value, L_AXLE_DIST=Lateral.xWheelbase.Value, LOOKAHEAD_GAIN_KPP=Lateral.Pursuit.kLookahead.Value, MIN_LOOKAHEAD_DIST=Lateral.Pursuit.xLookaheadMin.Value, MAX_LOOKAHEAD_DIST=Lateral.Pursuit.xLookaheadMax.Value, HEADING_WEIGHT_KH=Lateral.Pursuit.nWeightHeadingErr.Value}
      mask prompts: MAX_STEERING_ANGLE_DEG "Maximum steering angle (degrees)"; L_AXLE_DIST "Distance from the vehicle's reference point (currentPose) to the front axle (m)"; LOOKAHEAD_GAIN_KPP "Proportional gain for lookahead distance (Ld = K_pp * v_x)"; MIN_LOOKAHEAD_DIST "Minimum lookahead distance (m)"; MAX_LOOKAHEAD_DIST "Maximum lookahead distance (m)"; HEADING_WEIGHT_KH "Weight for the heading error term"
      mask help:
      | Implements PurePursuit method for lateral control.
      | Supports forward and reverse driving.
      | Pure Pursuit is based on Coulter, R. Craig. (1992). Implementation of the Pure Pursuit Path Tracking Algorithm. Carnegie Mellon University, The Robotics Institute. Technical Report CMU-RI-TR-92-01.
      mask DialogControl Container5 Prompt: Vehicle Parameters
      mask DialogControl Container4 Prompt: Pure Pursuit Method Parameters
  Stanley : Subsystem  VariantControl=Stanley  mask(Lateral Driver (Stanley)){MAX_STEERING_ANGLE_DEG=Lateral.aMaxSteer.Value, L_AXLE_DIST=Lateral.xWheelbase.Value, K_cte_forward=Lateral.Stanley.NForward.Value, K_cte_reverse=Lateral.Stanley.NReverse.Value}
      mask prompts: MAX_STEERING_ANGLE_DEG "Maximum steering angle (degrees)"; L_AXLE_DIST "Distance from the vehicle's reference point (currentPose) to the front axle (m)"; K_cte_forward "Cross-track error gain for forward"; K_cte_reverse "Cross-track error gain for reverse"
      mask help:
      | Implements Stanley method for lateral control.
      | Supports forward and reverse driving.
      | Stanley method is based on Hoffmann et al. (2007), "Autonomous Automobile Trajectory Tracking for Off-Road Driving"
      mask DialogControl Container5 Prompt: Vehicle Parameters
      mask DialogControl Container3 Prompt: Stanley Method Parameters
  steeringAngle : Outport

== system sm_car/Driver/Closed Loop/Driver/Longitudinal Driver ==
  Preview : Inport
  dir : Inport  Port=2
  vx : Inport  Port=3
  Distance : Inport  Port=4
  current_slope_rad : Inport  Port=5
  Braking : Subsystem
  Bus Selector3 : BusSelector  OutputSignals=pp_preview_dist_pts,pp_preview_speed_pts
  Constant1 : Constant  Value=mVehicle
  Constant10 : Constant  Value=KI_SPEED
  Constant11 : Constant  Value=MAX_ACCEL_MPS2
  Constant12 : Constant  Value=MAX_DECEL_MPS2
  Constant14 : Constant  Value=SPEED_LOOKAHEAD_TIME
  Constant3 : Constant  Value=gGravity
  Constant4 : Constant  Value=C_ROLLING_RESISTANCE_COEFF
  Constant6 : Constant  Value=FTractive
  Constant8 : Constant  Value=KP_SPEED
  Drag : Subsystem
  Integral Error : Integrator
  Longitudinal Driver : MATLAB Function  TreatAsAtomicUnit=on
  Saturation1 : Saturate  UpperLimit=1  LowerLimit=0  ZeroCross=off
  Saturation2 : Saturate  UpperLimit=1  LowerLimit=0  ZeroCross=off
  AccelCmd : Outport
  DecelCmd : Outport  Port=2
  wires:
  Braking/1(myu*g*m) -> Longitudinal Driver/13(MAX_NET_BRAKING_FORCE_N)
  Drag/1(0.5*Cd*rho*A) -> Longitudinal Driver/11(C_AERO_DRAG_COEFF)
  Constant12/1 -> Longitudinal Driver/17(MAX_DECEL_MPS2)
  dir/1 -> Longitudinal Driver/5(dir)
  Constant11/1 -> Longitudinal Driver/16(MAX_ACCEL_MPS2)
  current_slope_rad/1 -> Longitudinal Driver/6(current_slope_rad)
  Saturation2/1 -> DecelCmd/1  "rBrakePedal"
  Saturation1/1 -> AccelCmd/1  "rAccelPedal"
  Preview/1 -> Bus Selector3/1
  Longitudinal Driver/2(DecelCmd) -> Saturation2/1
  vx/1 -> Longitudinal Driver/4(current_vx)
  Constant8/1 -> Longitudinal Driver/14(KP_SPEED)
  Bus Selector3/2 -> Longitudinal Driver/2(pp_preview_speed_pts)  "<pp_preview_speed_pts>"
  Constant1/1 -> Longitudinal Driver/8(VEHICLE_MASS_KG)
  Constant4/1 -> Longitudinal Driver/10(C_ROLLING_RESISTANCE_COEFF)
  Constant14/1 -> Longitudinal Driver/7(SPEED_LOOKAHEAD_TIME)
  Integral Error/1 -> Longitudinal Driver/18(integral_error_input)
  Longitudinal Driver/3(v_error_out) -> Integral Error/1
  Constant3/1 -> Longitudinal Driver/9(GRAVITY_MPS2)
  Constant10/1 -> Longitudinal Driver/15(KI_SPEED)
  Longitudinal Driver/1(AccelCmd) -> Saturation1/1
  Distance/1 -> Longitudinal Driver/3(ad_vehicle)
  Bus Selector3/1 -> Longitudinal Driver/1(pp_preview_dist_pts)  "<pp_preview_dist_pts>"
  Constant6/1 -> Longitudinal Driver/12(MAX_NET_DRIVING_FORCE_N)

== system sm_car/Driver/Closed Loop/Driver/Ref Pose and Distance ==
  Ref : Inport
  Bus Selector : BusSelector  OutputSignals=x,y,ayaw,dist
  Mux : Mux  Inputs=3
  RefPose : Outport  VectorParamsAs1DForOutWhenUnconnected=off
  Dist : Outport  Port=2  VectorParamsAs1DForOutWhenUnconnected=off
  wires:
  Bus Selector/4 -> Dist/1  "<dist>"
  Bus Selector/1 -> Mux/1  "<x>"
  Ref/1 -> Bus Selector/1
  Mux/1 -> RefPose/1
  Bus Selector/2 -> Mux/2  "<y>"
  Bus Selector/3 -> Mux/3  "<ayaw>"

== system sm_car/Driver/Closed Loop/Driver Override/None ==
  In : Inport
  DrvBus : Outport
  wires:
  In/1 -> DrvBus/1

== system sm_car/Driver/Closed Loop/Driver Override/Override ==
  In : Inport
  Bus Creator5 : BusCreator  Inputs=4
  Bus Selector : BusSelector  OutputSignals=Reference,aSteerWheel,rAccelPedal,rBrakePedal
  Clock : Clock
  Compare To Constant : simulink/Logic and Bit Operations/Compare To Constant  relop=>=  const=Maneuver.TStart.aSteer.Value  OutDataTypeStr=boolean
  Compare To Constant1 : simulink/Logic and Bit Operations/Compare To Constant  relop=>=  const=Maneuver.TStart.rAccel.Value  OutDataTypeStr=boolean
  Compare To Constant2 : simulink/Logic and Bit Operations/Compare To Constant  relop=>=  const=Maneuver.TStart.rBrake.Value  OutDataTypeStr=boolean
  Input Sequence Accel Pedal : simulink/Sources/Repeating Sequence  rep_seq_t=Maneuver.Accel.t.Value  rep_seq_y=Maneuver.Accel.rPedal.Value
  Input Sequence Brake Pedal : simulink/Sources/Repeating Sequence  rep_seq_t=Maneuver.Brake.t.Value  rep_seq_y=Maneuver.Brake.rPedal.Value
  Input Sequence Steering Wheel : simulink/Sources/Repeating Sequence  rep_seq_t=Maneuver.Steer.t.Value  rep_seq_y=Maneuver.Steer.aWheel.Value
  Switch : Switch  Criteria=u2 > Threshold  SaturateOnIntegerOverflow=off  InputSameDT=off
  Switch1 : Switch  Criteria=u2 > Threshold  SaturateOnIntegerOverflow=off  InputSameDT=off
  Switch2 : Switch  Criteria=u2 > Threshold  SaturateOnIntegerOverflow=off  InputSameDT=off
  DrvBus : Outport
  wires:
  Input Sequence Brake Pedal/1 -> Switch2/1  "rBrakePedal"
  Input Sequence Accel Pedal/1 -> Switch1/1  "rAccelPedal"
  Input Sequence Steering Wheel/1 -> Switch/1  "aSteerWheel"
  Switch2/1 -> Bus Creator5/4  "rBrakePedal"
  Compare To Constant/1 -> Switch/2
  Clock/1 -> Compare To Constant/1, Compare To Constant1/1, Compare To Constant2/1
  Bus Selector/4 -> Switch2/3  "<rBrakePedal>"
  Switch1/1 -> Bus Creator5/3  "rAccelPedal"
  Bus Selector/3 -> Switch1/3  "<rAccelPedal>"
  Bus Selector/1 -> Bus Creator5/1  "<Reference>"
  Switch/1 -> Bus Creator5/2  "aSteerWheel"
  Bus Selector/2 -> Switch/3  "<aSteerWheel>"
  Bus Creator5/1 -> DrvBus/1  "DrvBus"
  In/1 -> Bus Selector/1
  Compare To Constant1/1 -> Switch1/2
  Compare To Constant2/1 -> Switch2/2

== system sm_car/Driver/Closed Loop/Maneuver/Count Lap ==
  note: If on the previous step, the vehicle was in the first 5 percent of the trajectory and now it is on the last 5 percent of the trajectory, decrement the number of laps.
  note: If on the previous step, the vehicle was in the last 5 percent of the trajectory and now it is on the first 5 percent of the trajectory, increment the number of laps.
  ad : Inport
  AND Add Lap : Logic  IconShape=distinctive  AllPortsSameDT=off  OutDataTypeStr=boolean
  AND Subtract Lap : Logic  IconShape=distinctive  AllPortsSameDT=off  OutDataTypeStr=boolean
  Data Type Conversion : DataTypeConversion  SaturateOnIntegerOverflow=off  RndMeth=Floor
  Data Type Conversion1 : DataTypeConversion  SaturateOnIntegerOverflow=off  RndMeth=Floor
  First 5 Percent : simulink/Logic and Bit Operations/Compare To Constant  relop=<=  const=max(Maneuver.Trajectory.xTrajectory.Value)*0.05  OutDataTypeStr=boolean  ZeroCross=off
  Last 5 Percent : simulink/Logic and Bit Operations/Compare To Constant  relop=>=  const=max(Maneuver.Trajectory.xTrajectory.Value)*0.95  OutDataTypeStr=boolean  ZeroCross=off
  Memory : Memory  InitialCondition=false
  Memory2 : Memory  InitialCondition=false
  OR : Logic  Operator=OR  IconShape=distinctive  AllPortsSameDT=off  OutDataTypeStr=boolean
  Sum : Sum  Inputs=+-|
  Triggered Subsystem : Subsystem  TreatAsAtomicUnit=on
  lapC : Outport  VectorParamsAs1DForOutWhenUnconnected=off
  wires:
  Sum/1 -> Triggered Subsystem/1(Up Down)  "Counter"
  AND Subtract Lap/1 -> Data Type Conversion1/1, OR/2  "Subtract Lap"
  AND Add Lap/1 -> OR/1, Data Type Conversion/1  "Add Lap"
  Memory2/1 -> AND Subtract Lap/1
  OR/1 -> Triggered Subsystem/Trigger  "Trigger"
  Memory/1 -> AND Add Lap/1
  First 5 Percent/1 -> AND Add Lap/2, Memory2/1  "First 5"
  Triggered Subsystem/1(Num Laps) -> lapC/1
  Last 5 Percent/1 -> Memory/1, AND Subtract Lap/2  "Last 5"
  ad/1 -> Last 5 Percent/1, First 5 Percent/1
  Data Type Conversion/1 -> Sum/1
  Data Type Conversion1/1 -> Sum/2
